simulink model "ADCS_Software_test"  (R2025b)
settings: Solver=VariableStepAuto  StartTime=0.0  StopTime=t0*1.5  FixedStep=0.1  MaxStep=0.1  RelTol=1e-3
values from neighbouring files (symbols this model uses):
  B = [1 0 0]    [parameters.m]
  h0 = [1 1 1]*0.5    [parameters.m]
  h_max = 1.47    [parameters.m]
  I_RW = 1    [parameters.m]
  k_desat = 1    [parameters.m]
  kd_detumble = 1    [parameters.m]
  kd_hold = 1    [parameters.m]
  kd_point = 20    [parameters.m]
  kd_slew_fast = 1    [parameters.m]
  kd_slew_slow = 1    [parameters.m]
  kd_spin = 0    [parameters.m]
  kp_hold = 1    [parameters.m]
  kp_point = 2    [parameters.m]
  kp_slew_fast = 1    [parameters.m]
  kp_slew_slow = 1    [parameters.m]
  kp_spin = 1    [parameters.m]
  omega_0 = [0 0 0.0011]    [parameters.m]
  omega_thr = 0.1    [parameters.m]    (also in run_ADCS_FSM_test_suite.m = 1)
  omega_zero = 0.001    [parameters.m]
  P = satellite_params()    [individual_test_with_dynamics.m]    (also in parameters.m; test.m = thrusters(:, 1:3))
  q0 = [sqrt(0.5) -sqrt(0.5) 0 0]    [parameters.m]
  ts = 0.1    [parameters.m]
undefined symbols (not defined in the file or in its folder): IAU
libraries: matrix_library x10, simulink x3, sim3dlib x2, aerolibutil x2, aerolibtransform2 x1
(part 1 of 2)
settings Model: Creator=ADMIN  LastModifiedBy=ADMIN
settings DataIOCC: ExternalInput=ds

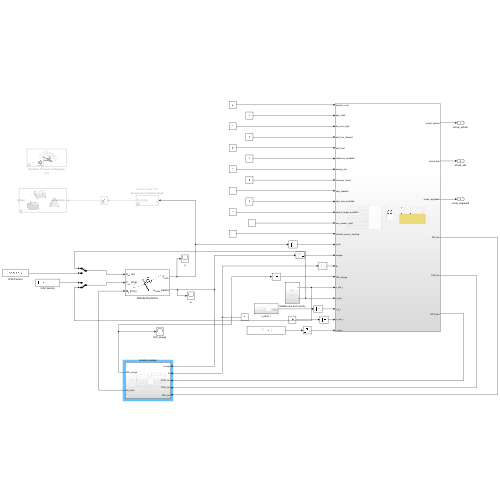
[thumbnail: Simulink's stored preview of the top-level diagram]
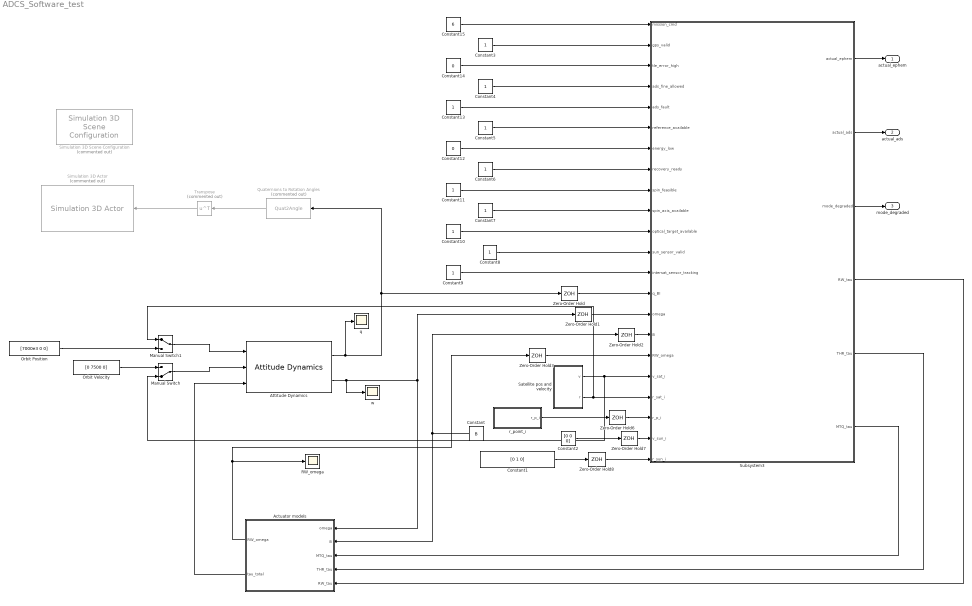
== system ADCS_Software_test ==
  Actuator models : Subsystem
  Attitude Dynamics : AttitudeDynamics  dateOut=off  mass=P.mass0  inertia=P.I0  outputFuelStatus=off  attitude=q0.'  attitudeRate=omega_0.'  useGravGrad=off  angleUnits=Radians
  Constant : Constant  Value=B
  Constant1 : Constant  Value=[0 1 0]
  Constant{3..11,13} (10 alike) : Constant  OutDataTypeStr=boolean
  Constant12 : Constant  Value=0  OutDataTypeStr=boolean
  Constant14 : Constant  Value=0  OutDataTypeStr=boolean
  Constant15 : Constant  Value=6  OutDataTypeStr=uint8
  Constant2 : Constant  Value=[0 0 0]
  Manual Switch : ManualSwitch  CurrentSetting=0
  Manual Switch1 : ManualSwitch
  Orbit Position : Constant  Value=[7000e3 0 0]
  Orbit Velocity : Constant  Value=[0 7500 0]
  Quaternions to Rotation Angles : Quat2Angle  Commented=on
      settings: AttributesFormatString=Rotation Order: %<rotationOrder>
  RW_omega : Scope
      settings: ActiveDisplayYMinimum=-1.8261016665257295  ActiveDisplayYMaximum=1.7349149987315644  DataLoggingVariableName=ScopeData5
  Satellite pos and velocity : Subsystem
  Simulation 3D Actor : sim3dlib/Simulation 3D Actor  Priority=1  Commented=on  ActorName=M4V  ParentName=Scene Origin  Operation=Create at setup  InitScriptText=|  SampleTime=-1  Translation=[0 0 0]  Rotation=[0 0 0]  Scale=[1 1 1]*0.1  InputsText=M4V.Rotation  aMode=5  ActorTag=M4V  ActorType=Sim3dActor  ID=C
      | % Reserved keywords:
      | % - Actor : handle to this actor object
      | % - World : handle to the world object
      | 
      | % Examples:
      | 
      | % Create a primitive geometry (optional)
      | % createShape(Actor, 'box', [1 1 1]);
      | 
      | % Initialize values (optional)
      | % Actor.Physics = true;
      | % Actor.Color = [1 0 0];
      | M4V.Mobility = sim3d.utils.MobilityTypes.Movable;
      | 
      | % For simple motion without gravity
      | M4V.Physics = true;
      | M4V.Gravity = false;
      | M4V.Collisions = false;
  Simulation 3D Scene Configuration : sim3dlib/Simulation 3D Scene Configuration  Priority=0  Commented=on  ProjectFormat=Default Scenes  SceneDesc=Space  ProjectName=C:\Program Files\MATLAB\R2025b\toolbox\shared\sim3d_projects\automotive_project_windows\UE\WindowsNoEditor\VehicleSimulation.exe  ScenePath=/Game/Maps/HwStrght  EnableOpenDRIVE=off  vehTagList={'Custom';'M4V';'Scene Origin'}  vehTag=Custom  AttachedCameraRelativeTranslation=[-20000 0 0]  FreeCameraDefaultInitialTranslation=[-6, 0, 2]  AttachedCameraRelativeRotation=[0 0 0]  FreeCameraDefaultInitialRotation=[0, -15, 0]  ViewpointName=Custom  FreeCameraInitialTranslation=[-1500 0 500]  ViewpointTranslation=[0 0 0]  FreeCameraInitialRotation=[0 0 0]  ViewpointRotation=[0 0 0]  OpVisEn=off  Ts=1  EnableWindow=on  EnableRemoteAccess=off  EnableWeather=off  SunAzimuth=90  SunAltitude=40.0  EnableGeospatialSun=off  Latitude=0  Longitude=0  Date=2023-01-01  Time=10:30:00  GeoTimeZone=-5.0  SunDaylightSaving=off  wind=0  clouds=10  EnableVolumetricClouds=off  CloudCoverage=0  CloudAltitude=6  fog=0  rain=0  RaindropsEffect=off  SnowDensity=0  EnableGeospatial=off  TilesetSource=Earth terrain  UseTrueOrigin=off  OriginHeight=200  OriginLatitude=40.744652  OriginLongitude=-73.988864  MapStyle=Aerial  AdditionalAssetIDs=[]  UseAdvancedSunSky=off  SolarTime=11  TimeZone=-5  Day=21  Month=9  Year=2022  UseDaylightSavingTime=on  DSTStartDay=10  DSTStartMonth=3  DSTEndDay=3  DSTEndMonth=11  DSTSwitchHour=2  sensorTag=MainCamera1  sensorId=1  sensorName=MainCamera1  mountLoc=Origin  offsetFlag=off  tmountOffset=[0, 0, 0]  rmountOffset=[0, 0, 0]  HorizontalResolution=1280  VerticalResolution=720  HorizontalFOV=60  mountPoint=[0 0 0]  mountOrientation=[0 0 0]  aMode=0  ID=1  GeoTrigger=Inactive  ViewNameList={'Custom'}  ViewTranslationList={'[-1500 0 500]'}  ViewRotationList={'[0 0 0]'}
      settings: AttributesFormatString=ICRF  LibrarySourceBlock=aerolibsim3d/Simulation 3D Scene Configuration
  Subsystem3 : Subsystem
  Transpose : Math  Commented=on  Operator=transpose
  Zero-Order Hold{,1..3,6..8} (7 alike) : ZeroOrderHold  SampleTime=ts
  q : Scope
      settings: ActiveDisplayYMinimum=-0.88388364004350628  ActiveDisplayYMaximum=0.88388494852608068  DataLoggingVariableName=ScopeData2
  r_point_i : Subsystem
  w : Scope
      settings: ActiveDisplayYMinimum=-0.03755798653451406  ActiveDisplayYMaximum=0.047606903153229088
  actual_ephem : Outport
  actual_ads : Outport  Port=2
  mode_degraded : Outport  Port=3
  wires:
  Constant13/1 -> Subsystem3/5(ads_fault)
  Constant3/1 -> Subsystem3/2(gps_valid)
  Constant15/1 -> Subsystem3/1(mission_cmd)
  Constant14/1 -> Subsystem3/3(tle_error_high)
  Constant4/1 -> Subsystem3/4(ads_fine_allowed)
  Constant5/1 -> Subsystem3/6(reference_available)
  Constant12/1 -> Subsystem3/7(energy_low)
  Constant6/1 -> Subsystem3/8(recovery_ready)
  Constant10/1 -> Subsystem3/11(optical_target_available)
  Constant7/1 -> Subsystem3/10(spin_axis_available)
  Constant11/1 -> Subsystem3/9(spin_feasible)
  Constant8/1 -> Subsystem3/12(sun_sensor_valid)
  Constant9/1 -> Subsystem3/13(intersat_sensor_tracking)
  Subsystem3/1(actual_ephem) -> actual_ephem/1
  Subsystem3/2(actual_ads) -> actual_ads/1
  Subsystem3/3(mode_degraded) -> mode_degraded/1
  Subsystem3/4(RW_tau) -> Actuator models/5(RW_tau)
  Actuator models/2(tau_total) -> Attitude Dynamics/3
  Subsystem3/5(THR_tau) -> Actuator models/4(THR_tau)
  Subsystem3/6(MTQ_tau) -> Actuator models/3(MTQ_tau)
  Transpose/1 -> Simulation 3D Actor/1
  Quaternions to Rotation Angles/1 -> Transpose/1
  Attitude Dynamics/2 -> w/1, Zero-Order Hold1/1, Actuator models/1(omega)
  Attitude Dynamics/1 -> q/1, Zero-Order Hold/1, Quaternions to Rotation Angles/1
  Constant/1 -> Zero-Order Hold2/1, Actuator models/2(B)
  Actuator models/1(RW_omega) -> Zero-Order Hold3/1, RW_omega/1
  r_point_i/1(r_p_i) -> Zero-Order Hold6/1
  Constant1/1 -> Zero-Order Hold8/1
  Constant2/1 -> Zero-Order Hold7/1
  Zero-Order Hold/1 -> Subsystem3/14(q_BI)
  Zero-Order Hold1/1 -> Subsystem3/15(omega)
  Zero-Order Hold2/1 -> Subsystem3/16(B)
  Zero-Order Hold3/1 -> Subsystem3/17(RW_omega)
  Satellite pos and velocity/1(v) -> Manual Switch/2, Subsystem3/18(v_sat_i)
  Satellite pos and velocity/2(r) -> Manual Switch1/1, Subsystem3/19(r_sat_i)
  Zero-Order Hold6/1 -> Subsystem3/20(r_p_i)
  Zero-Order Hold7/1 -> Subsystem3/21(v_sun_i)
  Zero-Order Hold8/1 -> Subsystem3/22(r_sun_i)
  Orbit Velocity/1 -> Manual Switch/1
  Manual Switch/1 -> Attitude Dynamics/2
  Manual Switch1/1 -> Attitude Dynamics/1
  Orbit Position/1 -> Manual Switch1/2

== system ADCS_Software_test/Actuator models ==
  omega : Inport
  B : Inport  Port=2
  MTQ_tau : Inport  Port=3
  THR_tau : Inport  Port=4
  RW_tau : Inport  Port=5
  Cross Product : matrix_library/Cross Product
  Gain : Gain  Gain=-1
  Gain1 : Gain  Gain=-1
  Gain2 : Gain  Gain=-1
  RW model : Subsystem
  Sum : Sum  Inputs=+++
  RW_omega : Outport
  tau_total : Outport  Port=2
  wires:
  omega/1 -> RW model/1(w)
  RW_tau/1 -> Gain1/1
  RW model/2(hw) -> RW_omega/1
  B/1 -> Cross Product/2
  MTQ_tau/1 -> Gain2/1
  Sum/1 -> tau_total/1
  Cross Product/1 -> Sum/1
  THR_tau/1 -> Gain/1
  RW model/1(tau) -> Sum/2
  Gain/1 -> Sum/3
  Gain1/1 -> RW model/2(tau_cmd)
  Gain2/1 -> Cross Product/1

== system ADCS_Software_test/Satellite pos and velocity ==
  Constant : Constant  Value=0
  Constant1 : Constant  Value=0
  Gain : Gain  Gain=-1
  Mux : Mux  Inputs=3
  Mux1 : Mux  Inputs=3
  Transpose : Math  Operator=transpose
  Transpose1 : Math  Operator=transpose
  cosine : Sin  Amplitude=7e6  Frequency=0.0011  Phase=pi/2  SampleTime=0
  cosine1 : Sin  Amplitude=7e6*0.0011  Frequency=0.0011  Phase=pi/2  SampleTime=0
  sine : Sin  Amplitude=7e6  Frequency=0.0011  SampleTime=0
  sine1 : Sin  Amplitude=7e6*0.0011  Frequency=0.0011  SampleTime=0
  v : Outport
  r : Outport  Port=2
  wires:
  sine/1 -> Mux/1
  cosine1/1 -> Mux1/1
  cosine/1 -> Mux/2
  Gain/1 -> Mux1/2
  Constant/1 -> Mux/3
  Constant1/1 -> Mux1/3
  sine1/1 -> Gain/1
  Mux/1 -> Transpose/1
  Transpose/1 -> r/1
  Mux1/1 -> Transpose1/1
  Transpose1/1 -> v/1

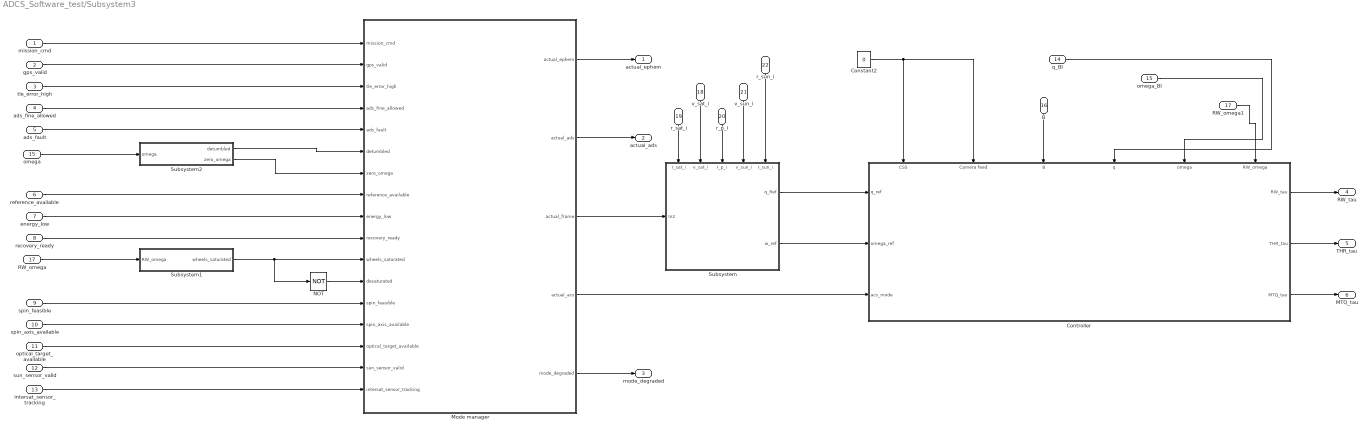
== system ADCS_Software_test/Subsystem3 ==
  mission_cmd : Inport
  gps_valid : Inport  Port=2
  tle_error_high : Inport  Port=3
  ads_fine_allowed : Inport  Port=4
  ads_fault : Inport  Port=5
  reference_available : Inport  Port=6
  energy_low : Inport  Port=7
  recovery_ready : Inport  Port=8
  spin_feasible : Inport  Port=9
  spin_axis_available : Inport  Port=10
  optical_target_available : Inport  Port=11
  sun_sensor_valid : Inport  Port=12
  intersat_sensor_tracking : Inport  Port=13
  q_BI : Inport  Port=14
  omega : Inport  Port=15
  B : Inport  Port=16
  RW_omega : Inport  Port=17
  v_sat_i : Inport  Port=18
  r_sat_i : Inport  Port=19
  r_p_i : Inport  Port=20
  v_sun_i : Inport  Port=21
  r_sun_i : Inport  Port=22
  Constant2 : Constant  Value=0
  Controller : Subsystem
      settings: PortSchema="{\"entries\":[{\"content\":{\"sides\":[{\"content\":{\"connectorIds\":[\"In1\",\"In2\",\"In3\"]},\"type\":\"ConnectorPlacement.EquallySpacedRectSide\",\"uuid\":\"3d0ce77c-a0dd-4e63-bb58-aa259872b360\"},{\"content\":{\"connectorIds\":[\"Out1\",\"Out2\",\"Out3\"],\"side\":\"RIGHT\"},\"type\":\"ConnectorPlacement.EquallySpacedRectSide\",\"uuid\":\"c51ce6d0-00d2-499a-9be1-102c03c9909c\"},{\"content\":{\"connectorIds\":[\"In4\",\"In5\",\"In6\",\"In7\",\"In8\",\"In9\"],\"side\":\"TOP\"},\"type\":\"ConnectorPlacement.EquallySpacedRectSide\",\"uuid\":\"ed1e7bc4-2cca-4611-893f-1128994bf2d9\"},{\"content\":{\"side\":\"BOTTOM\"},\"type\":\"ConnectorPlacement.EquallySpacedRectSide\",\"uuid\":\"574e7f6a-1005-4b0c-82f8-22f1ef6841a8\"}]},\"type\":\"ConnectorPlacement.EquallySpacedConnector\",\"uuid\":\"15c446ec-b512-4968-b865-507fd68d8b0b\"}],\"packageUris\":[\"http://schema.mathworks.com/mf0/Connector/R2020b\"],\"version\":\"1.0\"}"
  Mode manager : Subsystem
  NOT : Logic  Operator=NOT  IconShape=distinctive  AllPortsSameDT=off  OutDataTypeStr=boolean
  RW_omega1 : InportShadow  Port=17
  Subsystem : Subsystem
      settings: PortSchema="{\"entries\":[{\"content\":{\"sides\":[{\"content\":{\"connectorIds\":[\"In1\"]},\"type\":\"ConnectorPlacement.EquallySpacedRectSide\",\"uuid\":\"74bf1b15-53db-441c-9152-7c9ad8598452\"},{\"content\":{\"connectorIds\":[\"Out1\",\"Out2\"],\"side\":\"RIGHT\"},\"type\":\"ConnectorPlacement.EquallySpacedRectSide\",\"uuid\":\"e98e0885-3f20-4aa1-b3a1-f2c890def05c\"},{\"content\":{\"connectorIds\":[\"In2\",\"In3\",\"In4\",\"In5\",\"In6\"],\"side\":\"TOP\"},\"type\":\"ConnectorPlacement.EquallySpacedRectSide\",\"uuid\":\"f0898a47-7ae2-48e7-af8a-6d6327a5175a\"}]},\"type\":\"ConnectorPlacement.EquallySpacedConnector\",\"uuid\":\"b563a257-d36a-4c1e-a9df-51a9ac9caccd\"}],\"packageUris\":[\"http://schema.mathworks.com/mf0/Connector/R2020b\"],\"version\":\"1.0\"}"
  Subsystem1 : Subsystem
  Subsystem2 : Subsystem
  omega_BI : InportShadow  Port=15
  actual_ephem : Outport
  actual_ads : Outport  Port=2
  mode_degraded : Outport  Port=3
  RW_tau : Outport  Port=4
  THR_tau : Outport  Port=5
  MTQ_tau : Outport  Port=6
  wires:
  spin_axis_available/1 -> Mode manager/14(spin_axis_available)
  Controller/1(RW_tau) -> RW_tau/1
  Mode manager/1(actual_ephem) -> actual_ephem/1
  Mode manager/5(mode_degraded) -> mode_degraded/1
  Constant2/1 -> Controller/5(Camera feed), Controller/4(CSS)
  gps_valid/1 -> Mode manager/2(gps_valid)
  RW_omega/1 -> Subsystem1/1(RW_omega)
  Subsystem2/1(detumbled) -> Mode manager/6(detumbled)
  Mode manager/2(actual_ads) -> actual_ads/1
  tle_error_high/1 -> Mode manager/3(tle_error_high)
  Controller/3(MTQ_tau) -> MTQ_tau/1
  Mode manager/4(actual_acs) -> Controller/3(acs_mode)
  Subsystem1/1(wheels_saturated) -> NOT/1, Mode manager/11(wheels_saturated)
  sun_sensor_valid/1 -> Mode manager/16(sun_sensor_valid)
  recovery_ready/1 -> Mode manager/10(recovery_ready)
  NOT/1 -> Mode manager/12(desaturated)
  ads_fine_allowed/1 -> Mode manager/4(ads_fine_allowed)
  spin_feasible/1 -> Mode manager/13(spin_feasible)
  ads_fault/1 -> Mode manager/5(ads_fault)
  energy_low/1 -> Mode manager/9(energy_low)
  intersat_sensor_tracking/1 -> Mode manager/17(intersat_sensor_tracking)
  optical_target_available/1 -> Mode manager/15(optical_target_available)
  mission_cmd/1 -> Mode manager/1(mission_cmd)
  omega/1 -> Subsystem2/1(omega)
  reference_available/1 -> Mode manager/8(reference_available)
  Controller/2(THR_tau) -> THR_tau/1
  RW_omega1/1 -> Controller/9(RW_omega)
  omega_BI/1 -> Controller/8(omega)
  B/1 -> Controller/6(B)
  Mode manager/3(actual_frame) -> Subsystem/1(In2)
  Subsystem/1(q_Ref) -> Controller/1(q_ref)
  Subsystem/2(w_ref) -> Controller/2(omega_ref)
  v_sat_i/1 -> Subsystem/3(v_sat_i)
  r_sat_i/1 -> Subsystem/2(r_sat_i)
  r_p_i/1 -> Subsystem/4(r_p_i)
  v_sun_i/1 -> Subsystem/5(v_sun_i)
  r_sun_i/1 -> Subsystem/6(r_sun_i)
  Subsystem2/2(zero_omega) -> Mode manager/7(zero_omega)
  q_BI/1 -> Controller/7(q)

== system ADCS_Software_test/r_point_i ==
  Clock : Clock
  Constant1 : Constant  Value=[28.521693, 77.025165, 0]
  Constant3 : Constant  Value=0
  Constant4 : Constant  Value=37
  Constant5 : Constant  Value=[0 0]
  Constant6 : Constant  Value=[0 0]
  LLA to ECI Position : aerolibtransform2/LLA to ECI Position  red=IAU-2000/2006  year=2013  month=January  day=1  hour=0  min=0  sec=0  deltaT=Sec  errorflag=Error  extraparamflag=on  eunits=Metric (MKS)  earthmodel=WGS84  flat=1/298.257223563  eqradius=6378137
      settings: AttributesFormatString=%<red>
  r_p_i : Outport
  wires:
  Constant1/1 -> LLA to ECI Position/1
  Constant6/1 -> LLA to ECI Position/5
  Constant3/1 -> LLA to ECI Position/2
  Constant4/1 -> LLA to ECI Position/3
  Constant5/1 -> LLA to ECI Position/4
  LLA to ECI Position/1 -> r_p_i/1
  Clock/1 -> LLA to ECI Position/6

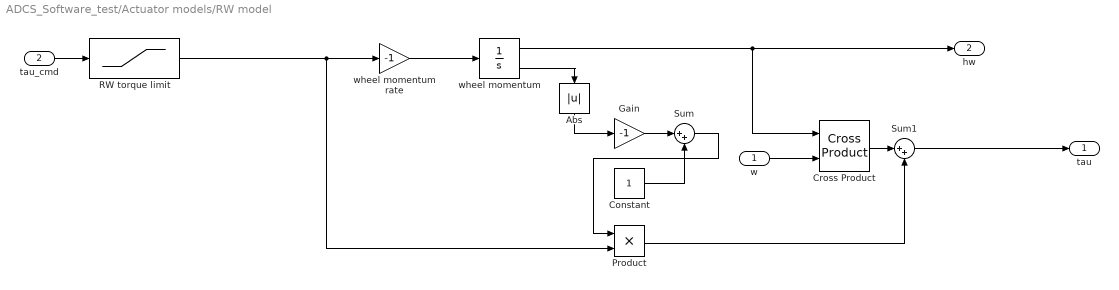
== system ADCS_Software_test/Actuator models/RW model ==
  w : Inport
  tau_cmd : Inport  Port=2
  Abs : Abs  SaturateOnIntegerOverflow=off
  Constant : Constant
  Cross Product : matrix_library/Cross Product
  Gain : Gain  Gain=-1
  Product : Product
  RW torque limit : Saturate  UpperLimit=P.rw.torque_max  LowerLimit=-P.rw.torque_max
  Sum : Sum  Inputs=|++
  Sum1 : Sum  Inputs=|++
  wheel momentum : Integrator  InitialCondition=h0  LimitOutput=on  UpperSaturationLimit=P.rw.h_max  LowerSaturationLimit=-P.rw.h_max  ShowSaturationPort=on
  wheel momentum rate : Gain  Gain=-1
  tau : Outport
  hw : Outport  Port=2
  wires:
  Abs/1 -> Gain/1
  wheel momentum rate/1 -> wheel momentum/1
  RW torque limit/1 -> Product/2, wheel momentum rate/1
  wheel momentum/1 -> Cross Product/1, hw/1
  wheel momentum/2 -> Abs/1
  Gain/1 -> Sum/1
  Constant/1 -> Sum/2
  Sum/1 -> Product/1
  tau_cmd/1 -> RW torque limit/1
  Product/1 -> Sum1/2
  w/1 -> Cross Product/2
  Cross Product/1 -> Sum1/1
  Sum1/1 -> tau/1

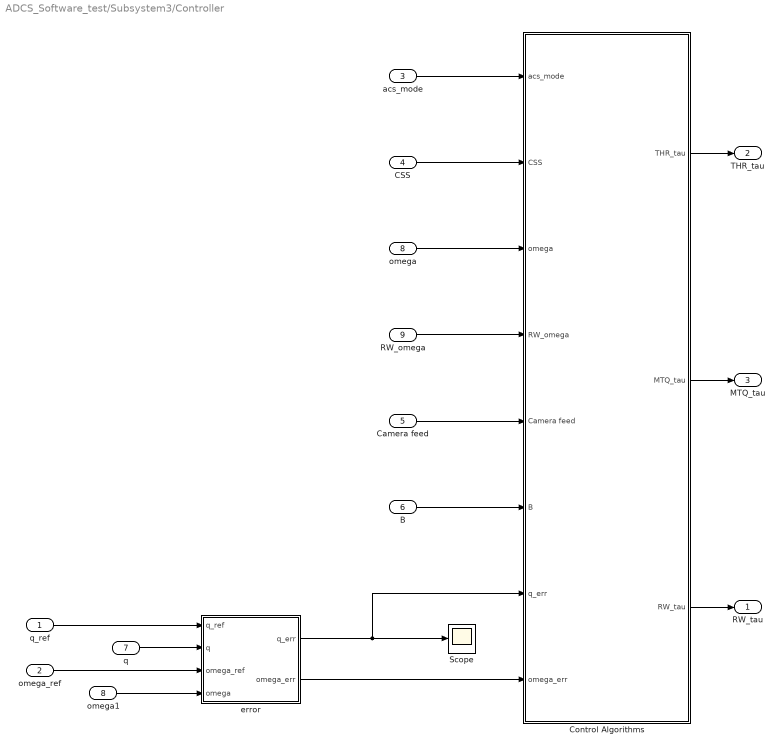
== system ADCS_Software_test/Subsystem3/Controller ==
  q_ref : Inport
  omega_ref : Inport  Port=2
  acs_mode : Inport  Port=3
  CSS : Inport  Port=4
  Camera feed : Inport  Port=5
  B : Inport  Port=6
  q : Inport  Port=7
  omega : Inport  Port=8
  RW_omega : Inport  Port=9
  Control Algorithms : Subsystem
  Scope : Scope
      settings: ActiveDisplayYMinimum=-1.1304178142300705  ActiveDisplayYMaximum=0.91127618067728278  DataLoggingVariableName=ScopeData8
  "error " : Subsystem
  omega1 : InportShadow  Port=8
  RW_tau : Outport
  THR_tau : Outport  Port=2
  MTQ_tau : Outport  Port=3
  wires:
  "error "/1(q_err) -> Scope/1, Control Algorithms/7(q_err)
  RW_omega/1 -> Control Algorithms/4(RW_omega)
  CSS/1 -> Control Algorithms/2(CSS)
  Camera feed/1 -> Control Algorithms/5(Camera feed)
  omega/1 -> Control Algorithms/3(omega)
  B/1 -> Control Algorithms/6(B)
  "error "/2(omega_err) -> Control Algorithms/8(omega_err)
  Control Algorithms/1(THR_tau) -> THR_tau/1
  Control Algorithms/2(MTQ_tau) -> MTQ_tau/1
  Control Algorithms/3(RW_tau) -> RW_tau/1
  q_ref/1 -> "error "/1(q_ref)
  q/1 -> "error "/2(q)
  omega_ref/1 -> "error "/3(omega_ref)
  omega1/1 -> "error "/4(omega)
  acs_mode/1 -> Control Algorithms/1(acs_mode)

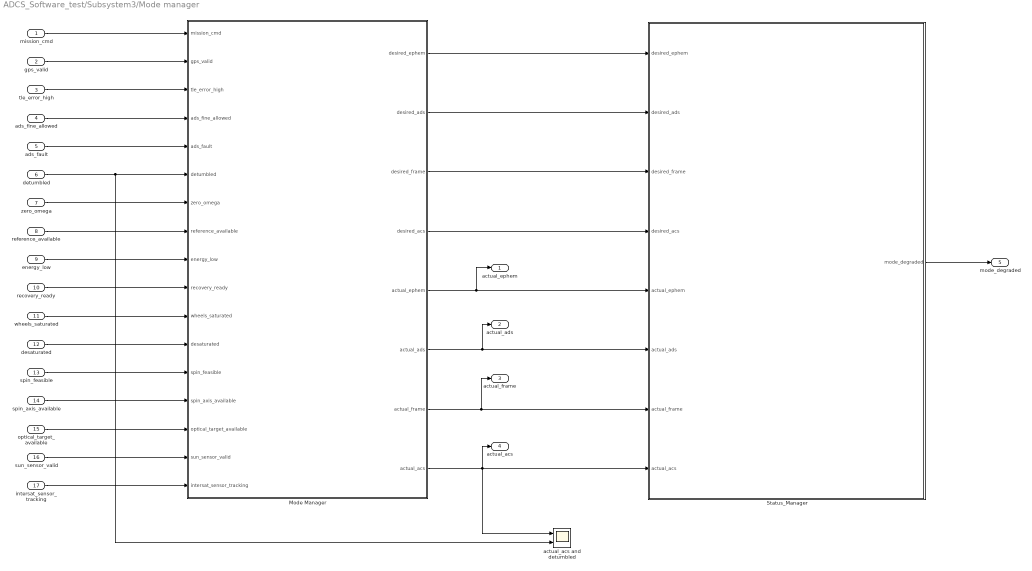
== system ADCS_Software_test/Subsystem3/Mode manager ==
  mission_cmd : Inport
  gps_valid : Inport  Port=2
  tle_error_high : Inport  Port=3
  ads_fine_allowed : Inport  Port=4
  ads_fault : Inport  Port=5
  detumbled : Inport  Port=6
  zero_omega : Inport  Port=7
  reference_available : Inport  Port=8
  energy_low : Inport  Port=9
  recovery_ready : Inport  Port=10
  wheels_saturated : Inport  Port=11
  desaturated : Inport  Port=12
  spin_feasible : Inport  Port=13
  spin_axis_available : Inport  Port=14
  optical_target_available : Inport  Port=15
  sun_sensor_valid : Inport  Port=16
  intersat_sensor_tracking : Inport  Port=17
  Mode Manager : Subsystem
  Status_Manager : Stateflow chart  TreatAsAtomicUnit=on
  actual_acs and detumbled : Scope  NumInputPorts=2
      settings: ActiveDisplayYMinimum=-0.74999999999999978  ActiveDisplayYMaximum=6.75  DataLoggingVariableName=ScopeData3
  actual_ephem : Outport
  actual_ads : Outport  Port=2
  actual_frame : Outport  Port=3
  actual_acs : Outport  Port=4
  mode_degraded : Outport  Port=5
  wires:
  recovery_ready/1 -> Mode Manager/10(recovery_ready)
  Mode Manager/2(desired_ads) -> Status_Manager/2(desired_ads)
  Mode Manager/8(actual_acs) -> actual_acs and detumbled/1, Status_Manager/8(actual_acs), actual_acs/1
  Mode Manager/1(desired_ephem) -> Status_Manager/1(desired_ephem)
  Mode Manager/5(actual_ephem) -> actual_ephem/1, Status_Manager/5(actual_ephem)
  Mode Manager/6(actual_ads) -> actual_ads/1, Status_Manager/6(actual_ads)
  Mode Manager/7(actual_frame) -> actual_frame/1, Status_Manager/7(actual_frame)
  Mode Manager/3(desired_frame) -> Status_Manager/3(desired_frame)
  Mode Manager/4(desired_acs) -> Status_Manager/4(desired_acs)
  reference_available/1 -> Mode Manager/8(reference_available)
  mission_cmd/1 -> Mode Manager/1(mission_cmd)
  ads_fault/1 -> Mode Manager/5(ads_fault)
  ads_fine_allowed/1 -> Mode Manager/4(ads_fine_allowed)
  wheels_saturated/1 -> Mode Manager/11(wheels_saturated)
  optical_target_available/1 -> Mode Manager/15(optical_target_available)
  detumbled/1 -> Mode Manager/6(detumbled), actual_acs and detumbled/2
  intersat_sensor_tracking/1 -> Mode Manager/17(intersat_sensor_tracking)
  desaturated/1 -> Mode Manager/12(desaturated)
  spin_feasible/1 -> Mode Manager/13(spin_feasible)
  tle_error_high/1 -> Mode Manager/3(tle_error_high)
  energy_low/1 -> Mode Manager/9(energy_low)
  Status_Manager/1(mode_degraded) -> mode_degraded/1
  spin_axis_available/1 -> Mode Manager/14(spin_axis_available)
  sun_sensor_valid/1 -> Mode Manager/16(sun_sensor_valid)
  gps_valid/1 -> Mode Manager/2(gps_valid)
  zero_omega/1 -> Mode Manager/7(zero_omega)

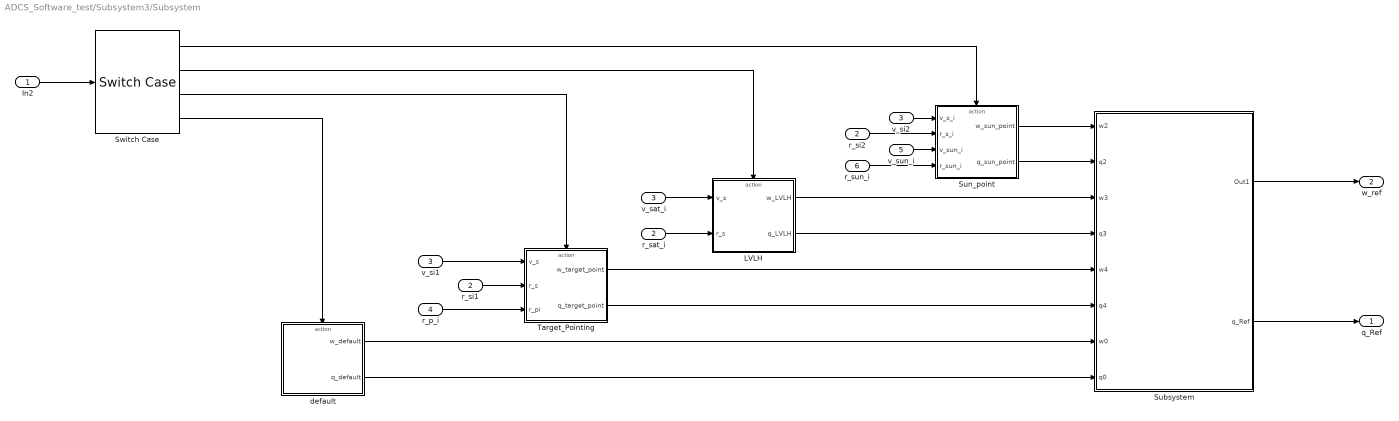
== system ADCS_Software_test/Subsystem3/Subsystem ==
  In2 : Inport
  r_sat_i : Inport  Port=2
  v_sat_i : Inport  Port=3
  r_p_i : Inport  Port=4
  v_sun_i : Inport  Port=5
  r_sun_i : Inport  Port=6
  LVLH : Subsystem
  Subsystem : Subsystem
  Sun_point : Subsystem
  Switch Case : SwitchCase  CaseConditions={2,3,4}
  Target_Pointing : Subsystem
  default : Subsystem
  r_si1 : InportShadow  Port=2
  r_si2 : InportShadow  Port=2
  v_si1 : InportShadow  Port=3
  v_si2 : InportShadow  Port=3
  q_Ref : Outport
  w_ref : Outport  Port=2
  wires:
  Switch Case/4 -> default/Action
  In2/1 -> Switch Case/1
  r_si1/1 -> Target_Pointing/2(r_s)
  v_si1/1 -> Target_Pointing/1(v_s)
  LVLH/1(w_LVLH) -> Subsystem/3(w3)
  LVLH/2(q_LVLH) -> Subsystem/4(q3)
  Target_Pointing/1(w_target_point) -> Subsystem/5(w4)
  Target_Pointing/2(q_target_point) -> Subsystem/6(q4)
  default/1(w_default) -> Subsystem/7(w0)
  default/2(q_default) -> Subsystem/8(q0)
  Subsystem/1(Out1) -> w_ref/1
  v_sat_i/1 -> LVLH/1(v_s)
  r_sat_i/1 -> LVLH/2(r_s)
  v_si2/1 -> Sun_point/1(v_s_i)
  r_si2/1 -> Sun_point/2(r_s_i)
  Sun_point/1(w_sun_point) -> Subsystem/1(w2)
  Sun_point/2(q_sun_point) -> Subsystem/2(q2)
  r_p_i/1 -> Target_Pointing/3(r_pi)
  v_sun_i/1 -> Sun_point/3(v_sun_i)
  r_sun_i/1 -> Sun_point/4(r_sun_i)
  Switch Case/1 -> Sun_point/Action
  Switch Case/2 -> LVLH/Action
  Switch Case/3 -> Target_Pointing/Action
  Subsystem/2(q_Ref) -> q_Ref/1

== system ADCS_Software_test/Subsystem3/Subsystem1 ==
  RW_omega : Inport
  Abs : Abs  SaturateOnIntegerOverflow=off
  Compare To Constant : simulink/Logic and Bit Operations/Compare To Constant  relop=>=  const=h_max  OutDataTypeStr=boolean
  Gain : Gain  Gain=I_RW
  Max of Elements : MinMax  Function=max
  wheels_saturated : Outport
  wires:
  Gain/1 -> Compare To Constant/1
  Abs/1 -> Max of Elements/1
  RW_omega/1 -> Abs/1
  Max of Elements/1 -> Gain/1
  Compare To Constant/1 -> wheels_saturated/1

== system ADCS_Software_test/Subsystem3/Subsystem2 ==
  omega : Inport
  Compare To Constant : simulink/Logic and Bit Operations/Compare To Constant  relop=<=  const=omega_thr^2  OutDataTypeStr=boolean
  Compare To Constant1 : simulink/Logic and Bit Operations/Compare To Constant  relop=<=  const=omega_zero^2  OutDataTypeStr=boolean
  Dot Product : DotProduct  OutDataTypeStr=Inherit: Inherit via internal rule
  detumbled : Outport
  zero_omega : Outport  Port=2
  wires:
  Compare To Constant/1 -> detumbled/1
  omega/1 -> Dot Product/2, Dot Product/1
  Dot Product/1 -> Compare To Constant1/1, Compare To Constant/1
  Compare To Constant1/1 -> zero_omega/1

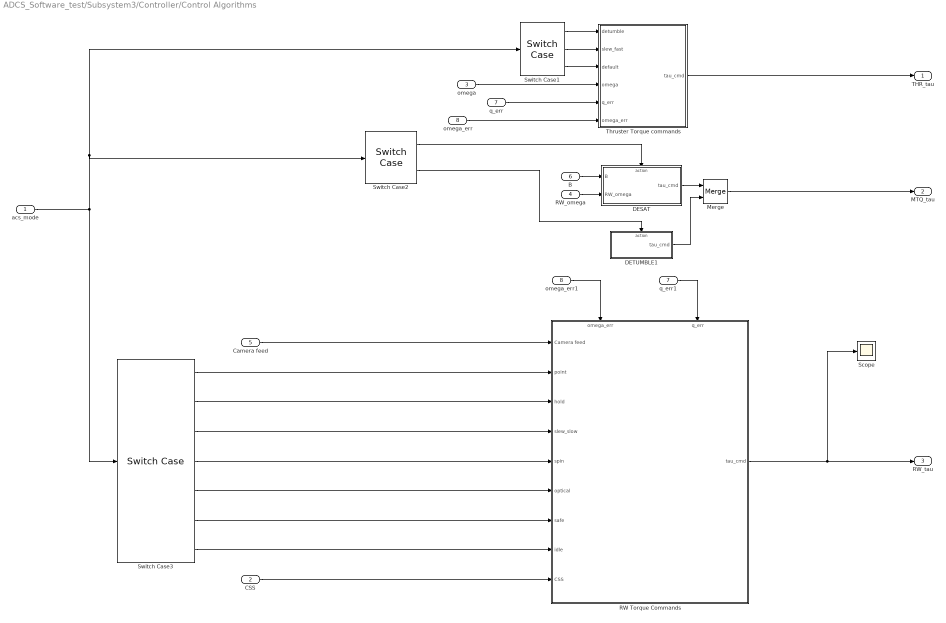
== system ADCS_Software_test/Subsystem3/Controller/Control Algorithms ==
  acs_mode : Inport
  CSS : Inport  Port=2
  omega : Inport  Port=3
  RW_omega : Inport  Port=4
  Camera feed : Inport  Port=5
  B : Inport  Port=6
  q_err : Inport  Port=7
  omega_err : Inport  Port=8
  DESAT : Subsystem  TreatAsAtomicUnit=on
  DETUMBLE1 : Subsystem  TreatAsAtomicUnit=on
  Merge : Merge
  RW Torque Commands : Subsystem
      settings: PortSchema="{\"entries\":[{\"content\":{\"sides\":[{\"content\":{\"connectorIds\":[\"In1\",\"In2\",\"In3\",\"In4\",\"In5\",\"In6\",\"In7\",\"In8\",\"In9\"]},\"type\":\"ConnectorPlacement.EquallySpacedRectSide\",\"uuid\":\"3d0ce77c-a0dd-4e63-bb58-aa259872b360\"},{\"content\":{\"connectorIds\":[\"Out1\"],\"side\":\"RIGHT\"},\"type\":\"ConnectorPlacement.EquallySpacedRectSide\",\"uuid\":\"c51ce6d0-00d2-499a-9be1-102c03c9909c\"},{\"content\":{\"connectorIds\":[\"In10\",\"In11\"],\"side\":\"TOP\"},\"type\":\"ConnectorPlacement.EquallySpacedRectSide\",\"uuid\":\"ed1e7bc4-2cca-4611-893f-1128994bf2d9\"}]},\"type\":\"ConnectorPlacement.EquallySpacedConnector\",\"uuid\":\"15c446ec-b512-4968-b865-507fd68d8b0b\"}],\"packageUris\":[\"http://schema.mathworks.com/mf0/Connector/R2020b\"],\"version\":\"1.0\"}"
  Scope : Scope
      settings: ActiveDisplayYMinimum=-6.5511260243979429E-17  ActiveDisplayYMaximum=6.5511160660656874E-17  DataLoggingVariableName=ScopeData7
  Switch Case1 : SwitchCase  CaseConditions={1,5}
  Switch Case2 : SwitchCase  CaseConditions={7}
  Switch Case3 : SwitchCase  CaseConditions={2,3,4,6,8,9}
  Thruster Torque commands : Subsystem
  omega_err1 : InportShadow  Port=8
  q_err1 : InportShadow  Port=7
  THR_tau : Outport
  MTQ_tau : Outport  Port=2
  RW_tau : Outport  Port=3
  wires:
  Camera feed/1 -> RW Torque Commands/1(Camera feed)
  RW_omega/1 -> DESAT/2(RW_omega)
  B/1 -> DESAT/1(B)
  RW Torque Commands/1(tau_cmd) -> Scope/1, RW_tau/1
  CSS/1 -> RW Torque Commands/9(CSS)
  Thruster Torque commands/1(tau_cmd) -> THR_tau/1
  omega/1 -> Thruster Torque commands/4(omega)
  omega_err/1 -> Thruster Torque commands/6(omega_err)
  q_err/1 -> Thruster Torque commands/5(q_err)
  omega_err1/1 -> RW Torque Commands/10(omega_err)
  q_err1/1 -> RW Torque Commands/11(q_err)
  Switch Case1/1 -> Thruster Torque commands/1(detumble)
  Switch Case1/2 -> Thruster Torque commands/2(slew_fast)
  Switch Case1/3 -> Thruster Torque commands/3(default)
  DETUMBLE1/1(tau_cmd) -> Merge/2
  Switch Case2/2 -> DETUMBLE1/Action
  DESAT/1(tau_cmd) -> Merge/1
  Merge/1 -> MTQ_tau/1
  Switch Case2/1 -> DESAT/Action
  Switch Case3/1 -> RW Torque Commands/2(point)
  Switch Case3/2 -> RW Torque Commands/3(hold)
  Switch Case3/3 -> RW Torque Commands/4(slew_slow)
  Switch Case3/4 -> RW Torque Commands/5(spin)
  Switch Case3/5 -> RW Torque Commands/6(optical)
  Switch Case3/6 -> RW Torque Commands/7(safe)
  Switch Case3/7 -> RW Torque Commands/8(idle)
  acs_mode/1 -> Switch Case3/1, Switch Case2/1, Switch Case1/1

== system ADCS_Software_test/Subsystem3/Controller/error  ==
  q_ref : Inport
  q : Inport  Port=2
  omega_ref : Inport  Port=3
  omega : Inport  Port=4
  Quaternion Inverse : aerolibutil/Quaternion Inverse
  Quaternion Multiplication : aerolibutil/Quaternion Multiplication
  Shortest q error : Switch  SaturateOnIntegerOverflow=off  InputSameDT=off
  Sum : Sum  Inputs=|+-
  q_err sign flip : Gain  Gain=-1
  split q_error : Demux  Outputs=[1 3]
  q_err : Outport
  omega_err : Outport  Port=2
  wires:
  q/1 -> Quaternion Inverse/1
  Sum/1 -> omega_err/1
  Quaternion Multiplication/1 -> split q_error/1
  q_ref/1 -> Quaternion Multiplication/2
  Quaternion Inverse/1 -> Quaternion Multiplication/1
  omega/1 -> Sum/1
  omega_ref/1 -> Sum/2
  Shortest q error/1 -> q_err/1
  split q_error/2 -> Shortest q error/1, q_err sign flip/1
  split q_error/1 -> Shortest q error/2
  q_err sign flip/1 -> Shortest q error/3

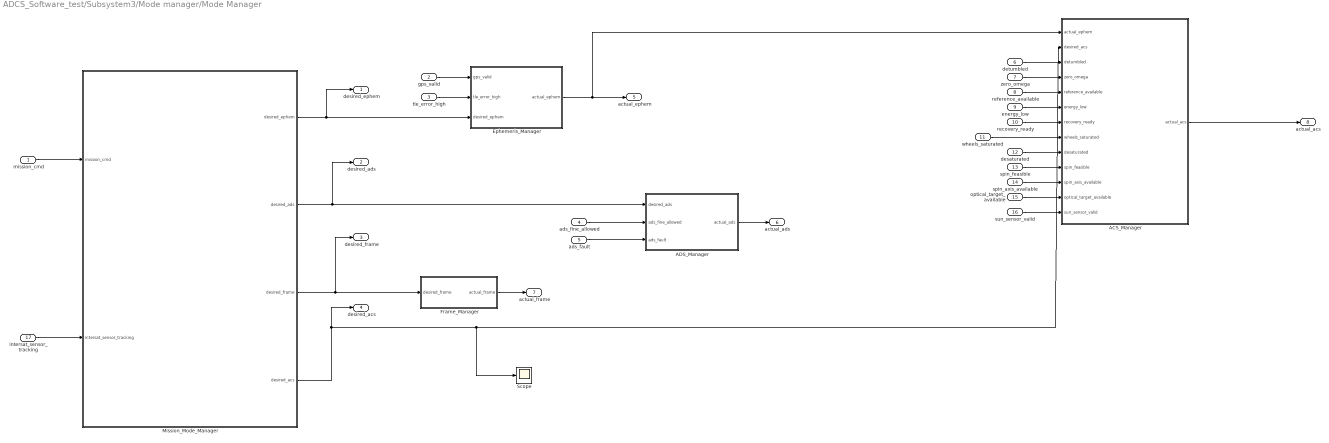
== system ADCS_Software_test/Subsystem3/Mode manager/Mode Manager ==
  mission_cmd : Inport  OutDataTypeStr=uint8  PortDimensions=1
  gps_valid : Inport  Port=2  OutDataTypeStr=boolean  PortDimensions=1
  tle_error_high : Inport  Port=3  OutDataTypeStr=boolean  PortDimensions=1
  ads_fine_allowed : Inport  Port=4  OutDataTypeStr=boolean  PortDimensions=1
  ads_fault : Inport  Port=5  OutDataTypeStr=boolean  PortDimensions=1
  detumbled : Inport  Port=6  OutDataTypeStr=boolean  PortDimensions=1
  zero_omega : Inport  Port=7
  reference_available : Inport  Port=8  OutDataTypeStr=boolean  PortDimensions=1
  energy_low : Inport  Port=9  OutDataTypeStr=boolean  PortDimensions=1
  recovery_ready : Inport  Port=10  OutDataTypeStr=boolean  PortDimensions=1
  wheels_saturated : Inport  Port=11  OutDataTypeStr=boolean  PortDimensions=1
  desaturated : Inport  Port=12  OutDataTypeStr=boolean  PortDimensions=1
  spin_feasible : Inport  Port=13  OutDataTypeStr=boolean  PortDimensions=1
  spin_axis_available : Inport  Port=14  OutDataTypeStr=boolean  PortDimensions=1
  optical_target_available : Inport  Port=15  OutDataTypeStr=boolean  PortDimensions=1
  sun_sensor_valid : Inport  Port=16  OutDataTypeStr=boolean  PortDimensions=1
  intersat_sensor_tracking : Inport  Port=17  OutDataTypeStr=boolean  PortDimensions=1
  ACS_Manager : Stateflow chart  TreatAsAtomicUnit=on
      settings: PortSchema="{\"entries\":[{\"content\":{\"sides\":[{\"content\":{\"connectorIds\":[\"In2\",\"In1\",\"In3\",\"In4\",\"In5\",\"In6\",\"In7\",\"In8\",\"In9\",\"In10\",\"In11\",\"In12\",\"In13\"]},\"type\":\"ConnectorPlacement.EquallySpacedRectSide\",\"uuid\":\"c64f5ed7-7a07-4761-a251-d625087249f8\"},{\"content\":{\"connectorIds\":[\"Out1\"],\"side\":\"RIGHT\"},\"type\":\"ConnectorPlacement.EquallySpacedRectSide\",\"uuid\":\"ff17dfa7-5a32-4799-bec0-131df3b46d45\"},{\"content\":{\"side\":\"TOP\"},\"type\":\"ConnectorPlacement.EquallySpacedRectSide\",\"uuid\":\"acaf274e-12ec-4fab-ab7e-ad580afcef6e\"}]},\"type\":\"ConnectorPlacement.EquallySpacedConnector\",\"uuid\":\"7d19de63-b993-417e-b6e9-9dc888da130b\"}],\"packageUris\":[\"http://schema.mathworks.com/mf0/Connector/R2020b\"],\"version\":\"1.0\"}"
  ADS_Manager : Stateflow chart  TreatAsAtomicUnit=on
  Ephemeris_Manager : Stateflow chart  TreatAsAtomicUnit=on
      settings: PortSchema="{\"entries\":[{\"content\":{\"sides\":[{\"content\":{\"connectorIds\":[\"In2\",\"In3\",\"In1\"]},\"type\":\"ConnectorPlacement.EquallySpacedRectSide\",\"uuid\":\"cbbccf67-8c60-498d-a98a-76db8747fb3a\"},{\"content\":{\"connectorIds\":[\"Out1\"],\"side\":\"RIGHT\"},\"type\":\"ConnectorPlacement.EquallySpacedRectSide\",\"uuid\":\"743b35d2-d398-4833-9c20-93b5e77612f2\"},{\"content\":{\"side\":\"TOP\"},\"type\":\"ConnectorPlacement.EquallySpacedRectSide\",\"uuid\":\"56075cc1-c683-438a-85bf-78d94186ffa6\"}]},\"type\":\"ConnectorPlacement.EquallySpacedConnector\",\"uuid\":\"bae867d4-09fc-4097-a23b-eff5fb3633ac\"}],\"packageUris\":[\"http://schema.mathworks.com/mf0/Connector/R2020b\"],\"version\":\"1.0\"}"
  Frame_Manager : Stateflow chart  TreatAsAtomicUnit=on
  Mission_Mode_Manager : Stateflow chart  TreatAsAtomicUnit=on
  Scope : Scope
      settings: ActiveDisplayYMinimum=-1  ActiveDisplayYMaximum=1  DataLoggingVariableName=ScopeData4
  desired_ephem : Outport
  desired_ads : Outport  Port=2
  desired_frame : Outport  Port=3
  desired_acs : Outport  Port=4
  actual_ephem : Outport  Port=5
  actual_ads : Outport  Port=6
  actual_frame : Outport  Port=7
  actual_acs : Outport  Port=8
  wires:
  sun_sensor_valid/1 -> ACS_Manager/13(sun_sensor_valid)
  ACS_Manager/1(actual_acs) -> actual_acs/1
  Mission_Mode_Manager/4(desired_acs) -> Scope/1, ACS_Manager/1(desired_acs), desired_acs/1
  energy_low/1 -> ACS_Manager/6(energy_low)
  Mission_Mode_Manager/1(desired_ephem) -> Ephemeris_Manager/1(desired_ephem), desired_ephem/1
  Frame_Manager/1(actual_frame) -> actual_frame/1
  optical_target_available/1 -> ACS_Manager/12(optical_target_available)
  Mission_Mode_Manager/2(desired_ads) -> desired_ads/1, ADS_Manager/1(desired_ads)
  tle_error_high/1 -> Ephemeris_Manager/3(tle_error_high)
  reference_available/1 -> ACS_Manager/5(reference_available)
  detumbled/1 -> ACS_Manager/3(detumbled)
  wheels_saturated/1 -> ACS_Manager/8(wheels_saturated)
  Mission_Mode_Manager/3(desired_frame) -> desired_frame/1, Frame_Manager/1(desired_frame)
  ADS_Manager/1(actual_ads) -> actual_ads/1
  ads_fine_allowed/1 -> ADS_Manager/2(ads_fine_allowed)
  Ephemeris_Manager/1(actual_ephem) -> actual_ephem/1, ACS_Manager/2(actual_ephem)
  gps_valid/1 -> Ephemeris_Manager/2(gps_valid)
  intersat_sensor_tracking/1 -> Mission_Mode_Manager/2(intersat_sensor_tracking)
  ads_fault/1 -> ADS_Manager/3(ads_fault)
  recovery_ready/1 -> ACS_Manager/7(recovery_ready)
  mission_cmd/1 -> Mission_Mode_Manager/1(mission_cmd)
  spin_axis_available/1 -> ACS_Manager/11(spin_axis_available)
  desaturated/1 -> ACS_Manager/9(desaturated)
  spin_feasible/1 -> ACS_Manager/10(spin_feasible)
  zero_omega/1 -> ACS_Manager/4(zero_omega)

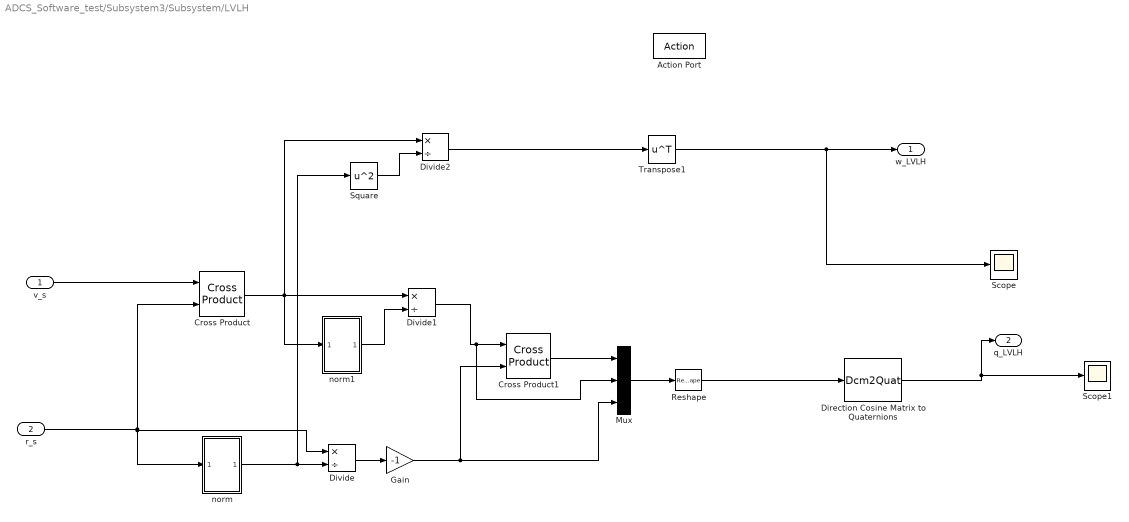
== system ADCS_Software_test/Subsystem3/Subsystem/LVLH ==
  v_s : Inport
  r_s : Inport  Port=2
  Action Port : ActionPort  ActionPortLabel=case [ 3 ]:
  Cross Product : matrix_library/Cross Product
  Cross Product1 : matrix_library/Cross Product
  Direction Cosine Matrix to Quaternions : Dcm2Quat
  Divide : Product  Inputs=*/
  Divide1 : Product  Inputs=*/
  Divide2 : Product  Inputs=*/
  Gain : Gain  Gain=-1
  Mux : Mux  Inputs=3
  Reshape : Reshape  OutputDimensionality=Customize  OutputDimensions=[3,3]
  Scope : Scope
      settings: ActiveDisplayYMinimum=-1  ActiveDisplayYMaximum=1  DataLoggingVariableName=ScopeData6
  Scope1 : Scope
      settings: ActiveDisplayYMinimum=-0.82867069291103368  ActiveDisplayYMaximum=0.87774872275294546
  Square : Math  Operator=square
  Transpose1 : Math  Operator=transpose
  norm : Subsystem
  norm1 : Subsystem
  w_LVLH : Outport
  q_LVLH : Outport  Port=2
  wires:
  Transpose1/1 -> Scope/1, w_LVLH/1
  Divide/1 -> Gain/1
  Divide1/1 -> Mux/2, Cross Product1/1
  norm1/1(Out1) -> Divide1/2
  Cross Product1/1 -> Mux/1
  Mux/1 -> Reshape/1
  Square/1 -> Divide2/2
  v_s/1 -> Cross Product/1
  r_s/1 -> norm/1(In1), Divide/1, Cross Product/2
  norm/1(Out1) -> Square/1, Divide/2
  Divide2/1 -> Transpose1/1
  Direction Cosine Matrix to Quaternions/1 -> Scope1/1, q_LVLH/1
  Gain/1 -> Mux/3, Cross Product1/2
  Cross Product/1 -> Divide2/1, Divide1/1, norm1/1(In1)
  Reshape/1 -> Direction Cosine Matrix to Quaternions/1

== system ADCS_Software_test/Subsystem3/Subsystem/Subsystem ==
  w2 : Inport
  q2 : Inport  Port=2
  w3 : Inport  Port=3
  q3 : Inport  Port=4
  w4 : Inport  Port=5
  q4 : Inport  Port=6
  w0 : Inport  Port=7
  q0 : Inport  Port=8
  Merge : Merge  Inputs=4
  Merge1 : Merge  Inputs=4
  Transpose2 : Math  Operator=transpose
  Out1 : Outport
  q_Ref : Outport  Port=2
  wires:
  q0/1 -> Merge1/4
  q4/1 -> Merge1/3
  q3/1 -> Merge1/2
  Merge/1 -> Transpose2/1
  q2/1 -> Merge1/1
  w0/1 -> Merge/4
  Merge1/1 -> q_Ref/1
  w4/1 -> Merge/3
  w3/1 -> Merge/2
  w2/1 -> Merge/1
  Transpose2/1 -> Out1/1

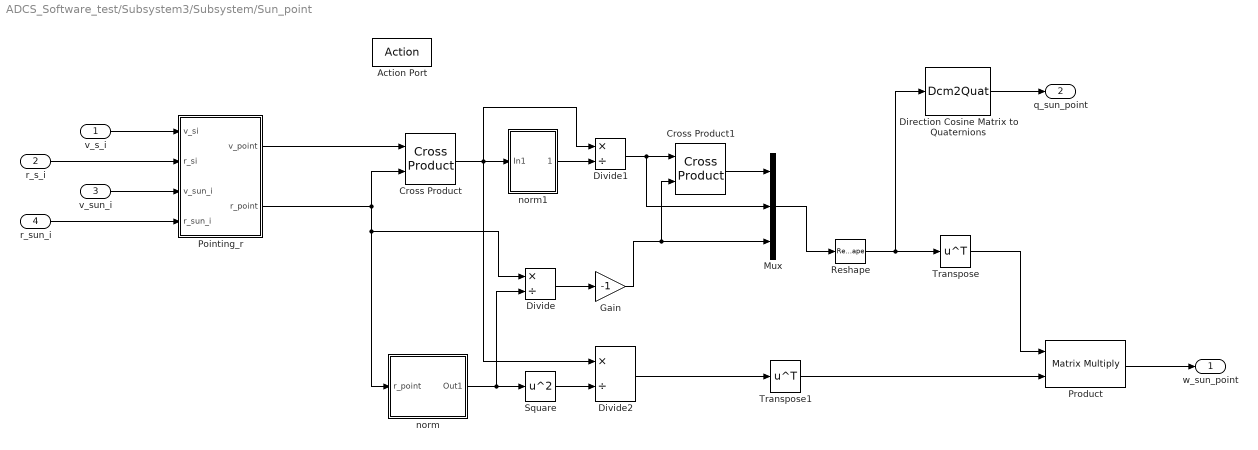
== system ADCS_Software_test/Subsystem3/Subsystem/Sun_point ==
  v_s_i : Inport
  r_s_i : Inport  Port=2
  v_sun_i : Inport  Port=3
  r_sun_i : Inport  Port=4
  Action Port : ActionPort  ActionPortLabel=case [ 2 ]:
  Cross Product : matrix_library/Cross Product
  Cross Product1 : matrix_library/Cross Product
  Direction Cosine Matrix to Quaternions : Dcm2Quat
  Divide : Product  Inputs=*/
  Divide1 : Product  Inputs=*/
  Divide2 : Product  Inputs=*/
  Gain : Gain  Gain=-1
  Mux : Mux  Inputs=3
  Pointing_r : Subsystem
  Product : Product  Multiplication=Matrix(*)
  Reshape : Reshape  OutputDimensionality=Customize  OutputDimensions=[3,3]
  Square : Math  Operator=square
  Transpose : Math  Operator=transpose
  Transpose1 : Math  Operator=transpose
  norm : Subsystem
  norm1 : Subsystem
  w_sun_point : Outport
  q_sun_point : Outport  Port=2
  wires:
  Product/1 -> w_sun_point/1
  Direction Cosine Matrix to Quaternions/1 -> q_sun_point/1
  Transpose/1 -> Product/1
  Reshape/1 -> Transpose/1, Direction Cosine Matrix to Quaternions/1
  Transpose1/1 -> Product/2
  Cross Product1/1 -> Mux/1
  Gain/1 -> Cross Product1/2, Mux/3
  Square/1 -> Divide2/2
  norm1/1(Out1) -> Divide1/2
  Divide1/1 -> Mux/2, Cross Product1/1
  Cross Product/1 -> norm1/1(In1), Divide1/1, Divide2/1
  Pointing_r/2(r_point) -> Divide/1, norm/1(r_point), Cross Product/2
  Mux/1 -> Reshape/1
  norm/1(Out1) -> Square/1, Divide/2
  Divide2/1 -> Transpose1/1
  Divide/1 -> Gain/1
  Pointing_r/1(v_point) -> Cross Product/1
  r_s_i/1 -> Pointing_r/2(r_si)
  v_s_i/1 -> Pointing_r/1(v_si)
  v_sun_i/1 -> Pointing_r/3(v_sun_i)
  r_sun_i/1 -> Pointing_r/4(r_sun_i)

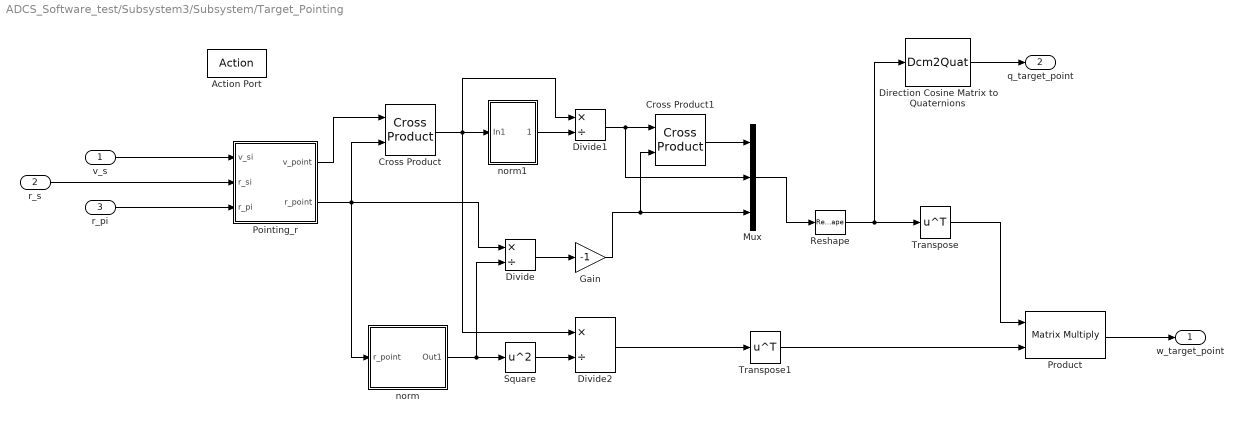
== system ADCS_Software_test/Subsystem3/Subsystem/Target_Pointing ==
  v_s : Inport
  r_s : Inport  Port=2
  r_pi : Inport  Port=3
  Action Port : ActionPort  ActionPortLabel=case [ 4 ]:
  Cross Product : matrix_library/Cross Product
  Cross Product1 : matrix_library/Cross Product
  Direction Cosine Matrix to Quaternions : Dcm2Quat
  Divide : Product  Inputs=*/
  Divide1 : Product  Inputs=*/
  Divide2 : Product  Inputs=*/
  Gain : Gain  Gain=-1
  Mux : Mux  Inputs=3
  Pointing_r : Subsystem
  Product : Product  Multiplication=Matrix(*)
  Reshape : Reshape  OutputDimensionality=Customize  OutputDimensions=[3,3]
  Square : Math  Operator=square
  Transpose : Math  Operator=transpose
  Transpose1 : Math  Operator=transpose
  norm : Subsystem
  norm1 : Subsystem
  w_target_point : Outport
  q_target_point : Outport  Port=2
  wires:
  v_s/1 -> Pointing_r/1(v_si)
  r_s/1 -> Pointing_r/2(r_si)
  Pointing_r/1(v_point) -> Cross Product/1
  Divide/1 -> Gain/1
  Divide2/1 -> Transpose1/1
  norm/1(Out1) -> Divide/2, Square/1
  Mux/1 -> Reshape/1
  Pointing_r/2(r_point) -> norm/1(r_point), Divide/1, Cross Product/2
  Cross Product/1 -> Divide2/1, Divide1/1, norm1/1(In1)
  Divide1/1 -> Cross Product1/1, Mux/2
  norm1/1(Out1) -> Divide1/2
  Square/1 -> Divide2/2
  Gain/1 -> Mux/3, Cross Product1/2
  Cross Product1/1 -> Mux/1
  Transpose1/1 -> Product/2
  Reshape/1 -> Direction Cosine Matrix to Quaternions/1, Transpose/1
  Transpose/1 -> Product/1
  Direction Cosine Matrix to Quaternions/1 -> q_target_point/1
  Product/1 -> w_target_point/1
  r_pi/1 -> Pointing_r/3(r_pi)

== system ADCS_Software_test/Subsystem3/Subsystem/default ==
  Action Port : ActionPort  ActionPortLabel=default:
  Constant : Constant  Value=[0; 0; 0]
  Constant1 : Constant  Value=[1 0 0 0]
  w_default : Outport
  q_default : Outport  Port=2
  wires:
  Constant1/1 -> q_default/1
  Constant/1 -> w_default/1

== system ADCS_Software_test/Subsystem3/Controller/Control Algorithms/DESAT ==
  B : Inport
  RW_omega : Inport  Port=2
  desat : ActionPort  ActionPortLabel=case [ 7 ]:
  Cross Product : matrix_library/Cross Product
  Divide : Product  Inputs=*/
  Dot Product : DotProduct  OutDataTypeStr=Inherit: Inherit via internal rule
  Gain : Gain  Gain=k_desat
  tau_cmd : Outport
  wires:
  B/1 -> Dot Product/1, Dot Product/2, Cross Product/2
  Divide/1 -> Gain/1
  Gain/1 -> tau_cmd/1
  Cross Product/1 -> Divide/1
  RW_omega/1 -> Cross Product/1
  Dot Product/1 -> Divide/2

== system ADCS_Software_test/Subsystem3/Controller/Control Algorithms/DETUMBLE1 ==
  detumble : ActionPort  ActionPortLabel=default:
  Constant : Constant  Value=[0 0 0]
  tau_cmd : Outport
  wires:
  Constant/1 -> tau_cmd/1

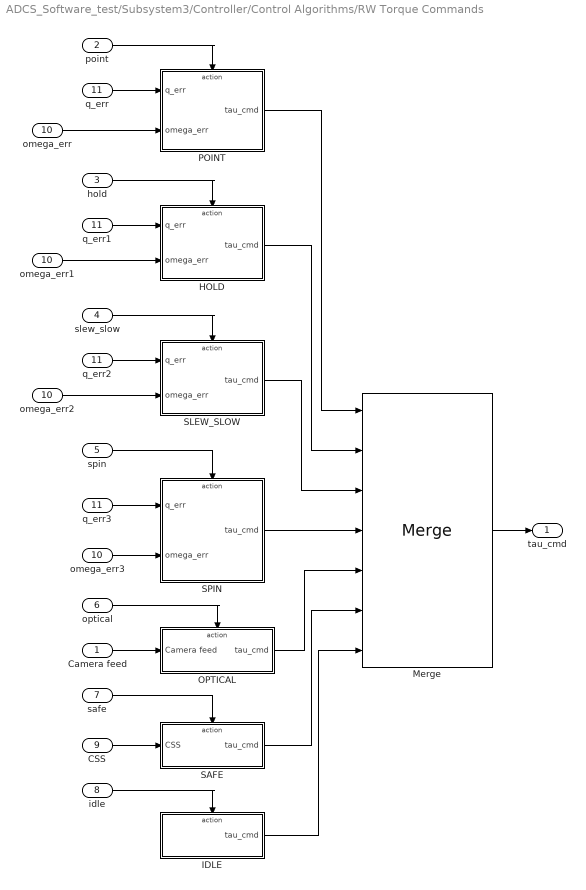
== system ADCS_Software_test/Subsystem3/Controller/Control Algorithms/RW Torque Commands ==
  Camera feed : Inport
  point : Inport  Port=2
  hold : Inport  Port=3
  slew_slow : Inport  Port=4
  spin : Inport  Port=5
  optical : Inport  Port=6
  safe : Inport  Port=7
  idle : Inport  Port=8
  CSS : Inport  Port=9
  omega_err : Inport  Port=10
  q_err : Inport  Port=11
  HOLD : Subsystem  TreatAsAtomicUnit=on
  IDLE : Subsystem  TreatAsAtomicUnit=on
  Merge : Merge  Inputs=7
  OPTICAL : Subsystem  TreatAsAtomicUnit=on
  POINT : Subsystem  TreatAsAtomicUnit=on
  SAFE : Subsystem  TreatAsAtomicUnit=on
  SLEW_SLOW : Subsystem  TreatAsAtomicUnit=on
  SPIN : Subsystem  TreatAsAtomicUnit=on
  omega_err1 : InportShadow  Port=10
  omega_err2 : InportShadow  Port=10
  omega_err3 : InportShadow  Port=10
  q_err1 : InportShadow  Port=11
  q_err2 : InportShadow  Port=11
  q_err3 : InportShadow  Port=11
  tau_cmd : Outport
  wires:
  safe/1 -> SAFE/Action
  slew_slow/1 -> SLEW_SLOW/Action
  hold/1 -> HOLD/Action
  SLEW_SLOW/1(tau_cmd) -> Merge/3
  point/1 -> POINT/Action
  q_err1/1 -> HOLD/1(q_err)
  omega_err/1 -> POINT/2(omega_err)
  q_err/1 -> POINT/1(q_err)
  omega_err1/1 -> HOLD/2(omega_err)
  q_err2/1 -> SLEW_SLOW/1(q_err)
  omega_err2/1 -> SLEW_SLOW/2(omega_err)
  spin/1 -> SPIN/Action
  omega_err3/1 -> SPIN/2(omega_err)
  optical/1 -> OPTICAL/Action
  Camera feed/1 -> OPTICAL/1(Camera feed)
  CSS/1 -> SAFE/1(CSS)
  idle/1 -> IDLE/Action
  POINT/1(tau_cmd) -> Merge/1
  HOLD/1(tau_cmd) -> Merge/2
  SPIN/1(tau_cmd) -> Merge/4
  OPTICAL/1(tau_cmd) -> Merge/5
  SAFE/1(tau_cmd) -> Merge/6
  IDLE/1(tau_cmd) -> Merge/7
  Merge/1 -> tau_cmd/1
  q_err3/1 -> SPIN/1(q_err)

== system ADCS_Software_test/Subsystem3/Controller/Control Algorithms/Thruster Torque commands ==
  detumble : Inport
  slew_fast : Inport  Port=2
  default : Inport  Port=3
  omega : Inport  Port=4
  q_err : Inport  Port=5
  omega_err : Inport  Port=6
  DEFAULT : Subsystem  TreatAsAtomicUnit=on
  DETUMBLE : Subsystem  TreatAsAtomicUnit=on
  Merge1 : Merge  Inputs=4
  SLEW_FAST : Subsystem  TreatAsAtomicUnit=on
  tau_cmd : Outport
  wires:
  SLEW_FAST/1(tau_cmd) -> Merge1/2
  omega/1 -> DETUMBLE/1(omega)
  DETUMBLE/1(tau_cmd) -> Merge1/1
  Merge1/1 -> tau_cmd/1
  q_err/1 -> SLEW_FAST/1(q_err)
  omega_err/1 -> SLEW_FAST/2(omega_err)
  slew_fast/1 -> SLEW_FAST/Action
  detumble/1 -> DETUMBLE/Action
  default/1 -> DEFAULT/Action
  DEFAULT/1(tau_cmd) -> Merge1/4

== system ADCS_Software_test/Subsystem3/Subsystem/LVLH/norm ==
  In1 : Inport
  Sqrt : Sqrt
  Square : Math  Operator=square
  Sum of Elements : Sum  Inputs=+
  Out1 : Outport
  wires:
  In1/1 -> Square/1
  Square/1 -> Sum of Elements/1
  Sum of Elements/1 -> Sqrt/1
  Sqrt/1 -> Out1/1

== system ADCS_Software_test/Subsystem3/Subsystem/LVLH/norm1 ==
  In1 : Inport
  Sqrt : Sqrt
  Square : Math  Operator=square
  Sum of Elements : Sum  Inputs=+
  Out1 : Outport
  wires:
  Sqrt/1 -> Out1/1
  Sum of Elements/1 -> Sqrt/1
  Square/1 -> Sum of Elements/1
  In1/1 -> Square/1

== system ADCS_Software_test/Subsystem3/Subsystem/Sun_point/Pointing_r ==
  v_si : Inport
  r_si : Inport  Port=2
  v_sun_i : Inport  Port=3
  r_sun_i : Inport  Port=4
  Sum : Sum  Inputs=|-+
  Sum1 : Sum  Inputs=|-+
  v_point : Outport
  r_point : Outport  Port=2
  wires:
  Sum1/1 -> v_point/1
  v_si/1 -> Sum1/1
  Sum/1 -> r_point/1
  r_si/1 -> Sum/1
  v_sun_i/1 -> Sum1/2
  r_sun_i/1 -> Sum/2

== system ADCS_Software_test/Subsystem3/Subsystem/Sun_point/norm ==
  r_point : Inport
  Sqrt : Sqrt
  Square : Math  Operator=square
  Sum of Elements : Sum  Inputs=+
  Out1 : Outport
  wires:
  r_point/1 -> Square/1
  Square/1 -> Sum of Elements/1
  Sum of Elements/1 -> Sqrt/1
  Sqrt/1 -> Out1/1

== system ADCS_Software_test/Subsystem3/Subsystem/Sun_point/norm1 ==
  In1 : Inport
  Sqrt : Sqrt
  Square : Math  Operator=square
  Sum of Elements : Sum  Inputs=+
  Out1 : Outport
  wires:
  Sqrt/1 -> Out1/1
  Sum of Elements/1 -> Sqrt/1
  Square/1 -> Sum of Elements/1
  In1/1 -> Square/1

== system ADCS_Software_test/Subsystem3/Subsystem/Target_Pointing/Pointing_r ==
  v_si : Inport
  r_si : Inport  Port=2
  r_pi : Inport  Port=3
  Sum : Sum  Inputs=-+|
  Sum1 : Sum  Inputs=|-+
  omega_E : Constant  Value=[0 0 7.2921159e-5]
  v_p : matrix_library/Cross Product
  v_point : Outport
  r_point : Outport  Port=2
  wires:
  r_si/1 -> Sum/1
  r_pi/1 -> v_p/2, Sum/2
  Sum/1 -> r_point/1
  v_si/1 -> Sum1/1
  omega_E/1 -> v_p/1
  Sum1/1 -> v_point/1
  v_p/1 -> Sum1/2

== system ADCS_Software_test/Subsystem3/Subsystem/Target_Pointing/norm ==
  r_point : Inport
  Sqrt : Sqrt
  Square : Math  Operator=square
  Sum of Elements : Sum  Inputs=+
  Out1 : Outport
  wires:
  Sqrt/1 -> Out1/1
  Sum of Elements/1 -> Sqrt/1
  Square/1 -> Sum of Elements/1
  r_point/1 -> Square/1

== system ADCS_Software_test/Subsystem3/Subsystem/Target_Pointing/norm1 ==
  In1 : Inport
  Sqrt : Sqrt
  Square : Math  Operator=square
  Sum of Elements : Sum  Inputs=+
  Out1 : Outport
  wires:
  In1/1 -> Square/1
  Square/1 -> Sum of Elements/1
  Sum of Elements/1 -> Sqrt/1
  Sqrt/1 -> Out1/1

== system ADCS_Software_test/Subsystem3/Controller/Control Algorithms/RW Torque Commands/HOLD ==
  q_err : Inport
  omega_err : Inport  Port=2
  hold : ActionPort  ActionPortLabel=case [ 3 ]:
  Gain : Gain  Gain=kd_hold
  Gain1 : Gain  Gain=kp_hold
  Sum : Sum  Inputs=|++
  tau_cmd : Outport
  wires:
  q_err/1 -> Gain1/1
  Gain1/1 -> Sum/1
  Sum/1 -> tau_cmd/1
  omega_err/1 -> Gain/1
  Gain/1 -> Sum/2

== system ADCS_Software_test/Subsystem3/Controller/Control Algorithms/RW Torque Commands/IDLE ==
  idle : ActionPort  ActionPortLabel=default:
  Constant : Constant  Value=[0 0 0]
  tau_cmd : Outport
  wires:
  Constant/1 -> tau_cmd/1

== system ADCS_Software_test/Subsystem3/Controller/Control Algorithms/RW Torque Commands/OPTICAL ==
  Camera feed : Inport
  optical : ActionPort  ActionPortLabel=case [ 8 ]:
  Constant : Constant  Value=[0 0 0]
  tau_cmd : Outport
  wires:
  Constant/1 -> tau_cmd/1

== system ADCS_Software_test/Subsystem3/Controller/Control Algorithms/RW Torque Commands/POINT ==
  q_err : Inport
  omega_err : Inport  Port=2
  point : ActionPort  ActionPortLabel=case [ 2 ]:
  Gain : Gain  Gain=kd_point
  Gain1 : Gain  Gain=-kp_point
  Sum : Sum  Inputs=|++
  tau_cmd : Outport
  wires:
  Sum/1 -> tau_cmd/1
  omega_err/1 -> Gain/1
  Gain1/1 -> Sum/1
  Gain/1 -> Sum/2
  q_err/1 -> Gain1/1

== system ADCS_Software_test/Subsystem3/Controller/Control Algorithms/RW Torque Commands/SAFE ==
  CSS : Inport
  safe : ActionPort  ActionPortLabel=case [ 9 ]:
  Constant : Constant  Value=[0 0 0]
  tau_cmd : Outport
  wires:
  Constant/1 -> tau_cmd/1

== system ADCS_Software_test/Subsystem3/Controller/Control Algorithms/RW Torque Commands/SLEW_SLOW ==
  q_err : Inport
  omega_err : Inport  Port=2
  slew_slow : ActionPort  ActionPortLabel=case [ 4 ]:
  Gain : Gain  Gain=kd_slew_slow
  Gain1 : Gain  Gain=kp_slew_slow
  Sum : Sum  Inputs=|++
  tau_cmd : Outport
  wires:
  Gain/1 -> Sum/2
  omega_err/1 -> Gain/1
  Sum/1 -> tau_cmd/1
  Gain1/1 -> Sum/1
  q_err/1 -> Gain1/1

== system ADCS_Software_test/Subsystem3/Controller/Control Algorithms/RW Torque Commands/SPIN ==
  q_err : Inport
  omega_err : Inport  Port=2
  spin : ActionPort  ActionPortLabel=case [ 6 ]:
  Constant : Constant  Value=[0 0 1]
  Constant1 : Constant  Value=[1 1 1]
  Gain : Gain  Gain=kd_spin
  Gain1 : Gain  Gain=kp_spin
  Gain2 : Gain  Gain=0.04
  Product : Product
  Sum : Sum  Inputs=|+-
  Sum1 : Sum  Inputs=|++
  Sum2 : Sum  Inputs=|+-
  tau_cmd : Outport
  wires:
  Sum/1 -> Gain/1
  omega_err/1 -> Sum/1
  Constant/1 -> Sum2/2, Gain2/1
  Gain/1 -> Sum1/2
  Sum1/1 -> tau_cmd/1
  Constant1/1 -> Sum2/1
  q_err/1 -> Product/1
  Sum2/1 -> Product/2
  Product/1 -> Gain1/1
  Gain1/1 -> Sum1/1
  Gain2/1 -> Sum/2

== system ADCS_Software_test/Subsystem3/Controller/Control Algorithms/Thruster Torque commands/DEFAULT ==
  default : ActionPort  ActionPortLabel=default:
  Constant : Constant  Value=[0 0 0]
  tau_cmd : Outport
  wires:
  Constant/1 -> tau_cmd/1

== system ADCS_Software_test/Subsystem3/Controller/Control Algorithms/Thruster Torque commands/DETUMBLE ==
  omega : Inport
  detumble : ActionPort  ActionPortLabel=case [ 1 ]:
  Gain : Gain  Gain=kd_detumble
  tau_cmd : Outport
  wires:
  omega/1 -> Gain/1
  Gain/1 -> tau_cmd/1

== system ADCS_Software_test/Subsystem3/Controller/Control Algorithms/Thruster Torque commands/SLEW_FAST ==
  q_err : Inport
  omega_err : Inport  Port=2
  slew_fast : ActionPort  ActionPortLabel=case [ 5 ]:
  Gain : Gain  Gain=kd_slew_fast
  Gain1 : Gain  Gain=kp_slew_fast
  Sum : Sum  Inputs=|++
  tau_cmd : Outport
  wires:
  Gain/1 -> Sum/2
  omega_err/1 -> Gain/1
  Sum/1 -> tau_cmd/1
  Gain1/1 -> Sum/1
  q_err/1 -> Gain1/1

== stateflow chart ADCS_Software_test/Subsystem3/Mode manager/Mode Manager/Frame_Manager ==
  state FRAME_INERTIAL
    entry:
    actual_frame = uint8(2);
  state FRAME_LVLH
    entry:
    actual_frame = uint8(3);
  state FRAME_BODY
    entry:
    actual_frame = uint8(1);
  state FRAME_EARTH_TARGET
    entry:
    actual_frame = uint8(4);
  state FRAME_IDLE
    entry:
    actual_frame = uint8(0);
  state FRAME_IMAGING_TDI
    entry:
    actual_frame = uint8(6);
  state FRAME_VNB
    entry:
    actual_frame = uint8(5);
  FRAME_INERTIAL -> (junction 11) : [desired_frame ~= uint8(2)]
  (junction 11) -> FRAME_INERTIAL [order 3] : [desired_frame == uint8(2)]
  FRAME_LVLH -> (junction 11) : [desired_frame ~= uint8(3)]
  (junction 11) -> FRAME_LVLH [order 4] : [desired_frame == uint8(3)]
  FRAME_BODY -> (junction 11) : [desired_frame ~= uint8(1)]
  (junction 11) -> FRAME_BODY [order 2] : [desired_frame == uint8(1)]
  FRAME_EARTH_TARGET -> (junction 11) : [desired_frame ~= uint8(4)]
  (junction 11) -> FRAME_EARTH_TARGET [order 5] : [desired_frame == uint8(4)]
  (junction 11) -> FRAME_IDLE [order 1] : [desired_frame == uint8(0)]
  FRAME_IDLE -> (junction 11) : [desired_frame ~= uint8(0)]
  FRAME_IMAGING_TDI -> (junction 11) : [desired_frame ~= uint8(6)]
  (junction 11) -> FRAME_VNB [order 6] : [desired_frame == uint8(5)]
  (junction 11) -> FRAME_IMAGING_TDI [order 7] : [desired_frame == uint8(6)]
  FRAME_VNB -> (junction 11) : [desired_frame ~= uint8(5)]
  (default) -> FRAME_IDLE
  data: desired_frame input uint8; actual_frame output uint8 =0
